simulink model "ElectricVehicleThermalManagementWithHeatPump"  (R2024b)
settings: Solver=VariableStepAuto  StartTime=0.0  StopTime=3600  RelTol=1e-3  AbsTol=1e-3
PreLoadFcn:
  | init_nmpc
InitFcn:
  | init_nmpc
model workspace: external: MATLAB File ElectricVehicleThermalManagementWithHeatPumpParameters.m (data not in the file)
values from neighbouring files (symbols this model uses):
  battery_C1_LUT = [1913.6 12447 30609 ... (first row only)    [ElectricVehicleThermalManagementWithHeatPumpParameters.m]
  battery_capacity_LUT = [280.081 276.25 276.392]    [ElectricVehicleThermalManagementWithHeatPumpParameters.m]
  battery_cell_cp = 795    [ElectricVehicleThermalManagementWithHeatPumpParameters.m]
  battery_cell_mass = 2.5    [ElectricVehicleThermalManagementWithHeatPumpParameters.m]
  battery_Em_LUT = [3.4966 3.5057 3.5148 ... (first row only)    [ElectricVehicleThermalManagementWithHeatPumpParameters.m]
  battery_N_cells = 20    [ElectricVehicleThermalManagementWithHeatPumpParameters.m]
  battery_Qe_init = 0    [ElectricVehicleThermalManagementWithHeatPumpParameters.m]
  battery_R0_LUT = [0.0117 0.0085 0.009 ... (first row only)    [ElectricVehicleThermalManagementWithHeatPumpParameters.m]
  battery_R1_LUT = [0.0109 0.0029 0.0013 ... (first row only)    [ElectricVehicleThermalManagementWithHeatPumpParameters.m]
  battery_SOC_LUT = [0; 0.1; 0.25; 0.5; 0.75; 0.9; 1]    [ElectricVehicleThermalManagementWithHeatPumpParameters.m]
  battery_T_init = -10    [ElectricVehicleThermalManagementWithHeatPumpParameters.m]
  battery_temperature_LUT = [5 20 40]    [ElectricVehicleThermalManagementWithHeatPumpParameters.m]
  cabin_duct_area = 0.04    [ElectricVehicleThermalManagementWithHeatPumpParameters.m]
  cabin_T_init = -10    [ElectricVehicleThermalManagementWithHeatPumpParameters.m]
  chiller_area_primary = 0.43982297150257105    (= 0.439822971503)    [ElectricVehicleThermalManagementWithHeatPumpParameters.m]
  chiller_N_baffles = 3    [ElectricVehicleThermalManagementWithHeatPumpParameters.m]
  chiller_N_tubes = 100    [ElectricVehicleThermalManagementWithHeatPumpParameters.m]
  chiller_tube_D = 0.0035    [ElectricVehicleThermalManagementWithHeatPumpParameters.m]
  chiller_tube_L = 0.4    [ElectricVehicleThermalManagementWithHeatPumpParameters.m]
  chiller_wall_conductivity = 240    [ElectricVehicleThermalManagementWithHeatPumpParameters.m]
  chiller_wall_thickness = 0.0001    [ElectricVehicleThermalManagementWithHeatPumpParameters.m]
  cond_evap_air_area_flow = 0.3906    [ElectricVehicleThermalManagementWithHeatPumpParameters.m]
  cond_evap_air_area_primary = 1.4834999999999998    (= 1.4835)    [ElectricVehicleThermalManagementWithHeatPumpParameters.m]
  cond_evap_W = 0.015    [ElectricVehicleThermalManagementWithHeatPumpParameters.m]
  cond_evap_wall_conductivity = 240    [ElectricVehicleThermalManagementWithHeatPumpParameters.m]
  cond_evap_wall_thickness = 0.0001    [ElectricVehicleThermalManagementWithHeatPumpParameters.m]
  coolant_channel_D = 0.0092    [ElectricVehicleThermalManagementWithHeatPumpParameters.m]
  coolant_pipe_D = 0.019    [ElectricVehicleThermalManagementWithHeatPumpParameters.m]
  coolant_T_init = -10    [ElectricVehicleThermalManagementWithHeatPumpParameters.m]
  coolant_tank_area = 0.0121    [ElectricVehicleThermalManagementWithHeatPumpParameters.m]
  coolant_tank_volume = 1.25    [ElectricVehicleThermalManagementWithHeatPumpParameters.m]
  coolant_valve_D_ratio_max = 0.95    [ElectricVehicleThermalManagementWithHeatPumpParameters.m]
  coolant_valve_D_ratio_min = 0.001    [ElectricVehicleThermalManagementWithHeatPumpParameters.m]
  coolant_valve_displacement = 0.0063    [ElectricVehicleThermalManagementWithHeatPumpParameters.m]
  coolant_valve_S_max = 0.0053    [ElectricVehicleThermalManagementWithHeatPumpParameters.m]
  evaporator_air_area_flow = 0.12    [ElectricVehicleThermalManagementWithHeatPumpParameters.m]
  evaporator_air_area_primary = 0.4323    [ElectricVehicleThermalManagementWithHeatPumpParameters.m]
  evaporator_W = 0.015    [ElectricVehicleThermalManagementWithHeatPumpParameters.m]
  evaporator_wall_conductivity = 240    [ElectricVehicleThermalManagementWithHeatPumpParameters.m]
  evaporator_wall_thickness = 0.0001    [ElectricVehicleThermalManagementWithHeatPumpParameters.m]
  expansion_valve_D_ratio_max = 0.9    [ElectricVehicleThermalManagementWithHeatPumpParameters.m]
  hex_area_primary = 0.070371675440411369    (= 0.0703716754404)    [ElectricVehicleThermalManagementWithHeatPumpParameters.m]
  hex_N_tubes = 64    [ElectricVehicleThermalManagementWithHeatPumpParameters.m]
  hex_tube_D = 0.0035    [ElectricVehicleThermalManagementWithHeatPumpParameters.m]
  hex_wall_conductivity = 240    [ElectricVehicleThermalManagementWithHeatPumpParameters.m]
  hex_wall_thickness = 0.0001    [ElectricVehicleThermalManagementWithHeatPumpParameters.m]
  inner_cond_air_area_flow = 0.1953    [ElectricVehicleThermalManagementWithHeatPumpParameters.m]
  inner_cond_air_area_primary = 0.99520000000000008    (= 0.9952)    [ElectricVehicleThermalManagementWithHeatPumpParameters.m]
  inner_cond_W = 0.02    [ElectricVehicleThermalManagementWithHeatPumpParameters.m]
  inner_cond_wall_conductivity = 240    [ElectricVehicleThermalManagementWithHeatPumpParameters.m]
  inner_cond_wall_thickness = 0.0001    [ElectricVehicleThermalManagementWithHeatPumpParameters.m]
  pump_speed_max = 1000    [ElectricVehicleThermalManagementWithHeatPumpParameters.m]
  radiator_air_area_flow = 0.097499999999999989    (= 0.0975)    [ElectricVehicleThermalManagementWithHeatPumpParameters.m]
  radiator_air_area_primary = 0.43687499999999996    (= 0.436875)    [ElectricVehicleThermalManagementWithHeatPumpParameters.m]
  radiator_W = 0.015    [ElectricVehicleThermalManagementWithHeatPumpParameters.m]
  radiator_wall_conductivity = 240    [ElectricVehicleThermalManagementWithHeatPumpParameters.m]
  radiator_wall_thickness = 0.0001    [ElectricVehicleThermalManagementWithHeatPumpParameters.m]
  refrigerant_p_init = 0.2    [ElectricVehicleThermalManagementWithHeatPumpParameters.m]
  refrigerant_pipe_D = 0.01    [ElectricVehicleThermalManagementWithHeatPumpParameters.m]
  refrigerant_valve_D_ratio_max = 0.95    [ElectricVehicleThermalManagementWithHeatPumpParameters.m]
  refrigerant_valve_displacement = 0.005    [ElectricVehicleThermalManagementWithHeatPumpParameters.m]
libraries: fl_lib x227, nesl_utility x162, SimscapeFluids_lib x30, LiBatteryElements_lib x16, slpidlib x3, SignalEditorBlockLib x1
(part 10 of 13)

== system ElectricVehicleThermalManagementWithHeatPump/Controls/Preview ==
  T_env : Inport
  Clock : Inport  Port=2
  Accleration : Constant  Value=|
      | [0
      | 0
      | 0
      | 0
      | 0
      | 0
      | 0
      | 0
      | 0
      | 0
      | 0
      | 0
      | 0
      | 0
      | 0
      | 4
      | 4
      | 1
      | 3
      | 2.50000000000000
      | 0.500000000000000
      | 0
      | 0
      | 0
      | 0
      | -0.500000000000000
      | -0.500000000000000
      | -1
      | -7
      | -6
      | 0
      | 0
      | 0
      | 0
      | 0
      | 0
      | 0
      | 0
      | 0
      | 0
      | 0
      | 0
      | 0
      | 0
      | 0
      | 0
      | 0
      | 0
      | 0
      | 0
      | 0
      | 0
      | 4
      | 4
      | 0
      | 1
      | 2.50000000000000
      | 2.50000000000000
      | 0.666666666666667
      | 1
      | 3.50000000000000
      | 4.50000000000000
      | 3
      | 2
      | 2
      | 0.500000000000000
      | 0
      | 0
      | 0
      | 0
      | 0
      | 0
      | 0
      | 0
      | 0
      | 0
      | 0
      | 0
      | 0
      | 0
      | 0
      | 0
      | -0.500000000000000
      | -0.500000000000000
      | 0
      | 0
      | 0
      | -0.500000000000000
      | -1.50000000000000
      | -2
      | -2.50000000000000
      | -2.50000000000000
      | -2.50000000000000
      | -2.50000000000000
      | -1.50000000000000
      | -8
      | -7.50000000000000
      | 0
      | 0
      | 0
      | 0
      | 0
      | 0
      | 0
      | 0
      | 0
      | 0
      | 0
      | 0
      | 0
      | 0
      | 0
      | 0
      | 0
      | 0
      | 0
      | 0
      | 0
      | 0
      | 3.50000000000000
      | 4
      | 0.500000000000000
      | 1
      | 3
      | 2.50000000000000
      | 0.333333333333333
      | 0.666666666666667
      | 2.50000000000000
      | 2.50000000000000
      | 2.50000000000000
      | 2.50000000000000
      | 2.50000000000000
      | 2
      | 1.50000000000000
      | 1.50000000000000
      | 1
      | 0.500000000000000
      | 1
      | 2.50000000000000
      | 2.50000000000000
      | 2
      | 1.50000000000000
      | 1.50000000000000
      | 1.50000000000000
      | 1
      | 1
      | 0.500000000000000
      | 0
      | 0
      | 0
      | 0
      | -0.500000000000000
      | -0.500000000000000
      | 0
      | 0
      | 0
      | -0.500000000000000
      | -1
      | -1.50000000000000
      | -2
      | -1.50000000000000
      | -1.50000000000000
      | -1.50000000000000
      | -1.50000000000000
      | -2
      | -0.500000000000000
      | 0
      | -0.500000000000000
      | 0
      | 0
      | 0
      | 0
      | 0
      | 0
      | 0
      | 0
      | 0
      | -0.666666666666667
      | -1
      | -2
      | -3
      | -3
      | -3
      | -3
      | -10
      | -8.50000000000000
      | 0
      | 0
      | 0
      | 0
      | 0
      | 0
      | 0
      | 0
      | 0
      | 0
      | 0
      | 0
      | 0
      | 0
      | 0
      | 0
      | 0
      | 0
      | 0
      | 0
      | 3
      | 4
      | 1
      | 1
      | 3
      | 2.50000000000000
      | 0.500000000000000
      | 0
      | 0
      | 0
      | 0
      | -0.500000000000000
      | -0.500000000000000
      | -1
      | -7
      | -6
      | 0
      | 0
      | 0
      | 0
      | 0
      | 0
      | 0
      | 0
      | 0
      | 0
      | 0
      | 0
      | 0
      | 0
      | 0
      | 0
      | 0
      | 0
      | 0
      | 0
      | 0
      | 0
      | 3
      | 4
      | 1
      | 1
      | 3
      | 2.50000000000000
      | 0.500000000000000
      | -0.500000000000000
      | 1.50000000000000
      | 4
      | 4
      | 3.50000000000000
      | 2.50000000000000
      | 1.50000000000000
      | 0.500000000000000
      | 0
      | 0
      | 0
      | 0
      | 0
      | 0
      | 0
      | 0
      | 0
      | 0
      | 0
      | 0
      | 0
      | 0
      | 0
      | 0
      | 0
      | -0.500000000000000
      | -0.500000000000000
      | 0
      | 0
      | -0.500000000000000
      | -1.50000000000000
      | -2
      | -2.50000000000000
      | -2.50000000000000
      | -2.50000000000000
      | -3
      | -9
      | -7.50000000000000
      | 0
      | 0
      | 0
      | 0
      | 0
      | 0
      | 0
      | 0
      | 0
      | 0
      | 0
      | 0
      | 0
      | 0
      | 0
      | 0
      | 0
      | 0
      | 0
      | 0
      | 0
      | 0
      | 0
      | 3
      | 3.50000000000000
      | 1
      | 1.50000000000000
      | 2.50000000000000
      | 2.50000000000000
      | 1.50000000000000
      | -0.500000000000000
      | 0.500000000000000
      | 3
      | 3
      | 2.50000000000000
      | 2
      | 2.50000000000000
      | 2.50000000000000
      | 2
      | 1
      | 0.333333333333333
      | 1
      | 2
      | 2
      | 2
      | 2
      | 1.50000000000000
      | 1.50000000000000
      | 1.50000000000000
      | 1
      | 0.500000000000000
      | 0
      | 0
      | 0
      | -0.500000000000000
      | 0
      | 0.500000000000000
      | -0.500000000000000
      | -0.500000000000000
      | 0
      | 0
      | -1
      | -2
      | -1.50000000000000
      | -1.50000000000000
      | -2
      | -2
      | -1.50000000000000
      | -1.50000000000000
      | -0.500000000000000
      | 0
      | -0.500000000000000
      | 0
      | 0
      | 0
      | 0
      | 0
      | 0
      | 0
      | 0
      | 0
      | -0.666666666666667
      | -1
      | -2
      | -3
      | -3
      | -3
      | -3
      | -10
      | -8.50000000000000
      | 0
      | 0
      | 0
      | 0
      | 0
      | 0
      | 0
      | 0
      | 0
      | 0
      | 0
      | 0
      | 0
      | 0
      | 0
      | 0
      | 0
      | 0
      | 0
      | 0
      | 3
      | 4
      | 1
      | 1
      | 3
      | 2.50000000000000
      | 0.500000000000000
      | 0
      | 0
      | 0
      | 0
      | -0.500000000000000
      | -0.500000000000000
      | -1
      | -7
      | -6
      | 0
      | 0
      | 0
      | 0
      | 0
      | 0
      | 0
      | 0
      | 0
      | 0
      | 0
      | 0
      | 0
      | 0
      | 0
      | 0
      | 0
      | 0
      | 0
      | 0
      | 0
      | 0
      | 3
      | 4
      | 1
      | 1
      | 2.50000000000000
      | 2.50000000000000
      | 1
      | -0.500000000000000
      | 1.50000000000000
      | 4.50000000000000
      | 4
      | 3
      | 2.50000000000000
      | 1.50000000000000
      | 0.500000000000000
      | 0
      | 0
      | 0
      | 0
      | 0
      | 0
      | 0
      | 0
      | 0
      | 0
      | 0
      | 0
      | 0
      | 0
      | 0
      | -0.500000000000000
      | 0
      | 0
      | -0.500000000000000
      | 0
      | 0
      | -0.500000000000000
      | -1.50000000000000
      | -2
      | -2.50000000000000
      | -2.50000000000000
      | -2.50000000000000
      | -3
      | -9
      | -7.50000000000000
      | 0
      | 0
      | 0
      | 0
      | 0
      | 0
      | 0
      | 0
      | 0
      | 0
      | 0
      | 0
      | 0
      | 0
      | 0
      | 0
      | 0
      | 0
      | 0
      | 0
      | 0
      | 0
      | 0
      | 3
      | 4
      | 1
      | 1
      | 2.50000000000000
      | 2.50000000000000
      | 1
      | 0
      | 1
      | 2
      | 3
      | 3
      | 2
      | 2
      | 2.50000000000000
      | 2.50000000000000
      | 1
      | 0.333333333333333
      | 1.33333333333333
      | 2.50000000000000
      | 2
      | 1.50000000000000
      | 1.50000000000000
      | 2
      | 1.50000000000000
      | 1
      | 1
      | 0.500000000000000
      | 0
      | 0
      | 0
      | 0
      | 0
      | -0.500000000000000
      | -0.500000000000000
      | 0
      | 0
      | 0
      | -1
      | -2
      | -1.50000000000000
      | -1.50000000000000
      | -2
      | -2
      | -1.50000000000000
      | -1.50000000000000
      | -1
      | 0
      | 0
      | 0
      | 0
      | 0
      | 0
      | 0
      | 0
      | 0
      | 0
      | 0
      | -0.666666666666667
      | -1
      | -2
      | -3
      | -3
      | -3
      | -3.50000000000000
      | -10
      | -8
      | 0
      | 0
      | 0
      | 0
      | 0
      | 0
      | 0
      | 0
      | 0
      | 0
      | 0
      | 0
      | 0
      | 0
      | 0
      | 0
      | 0
      | 0
      | 0
      | 0
      | 3
      | 4
      | 1
      | 1
      | 3
      | 2.50000000000000
      | 0.500000000000000
      | 0
      | 0
      | 0
      | 0
      | -0.500000000000000
      | -0.500000000000000
      | -1
      | -7
      | -6
      | 0
      | 0
      | 0
      | 0
      | 0
      | 0
      | 0
      | 0
      | 0
      | 0
      | 0
      | 0
      | 0
      | 0
      | 0
      | 0
      | 0
      | 0
      | 0
      | 0
      | 0
      | 0
      | 3
      | 4
      | 1
      | 1
      | 3
      | 2.50000000000000
      | 1
      | -0.500000000000000
      | 1
      | 4.50000000000000
      | 4
      | 3
      | 2.50000000000000
      | 1.50000000000000
      | 0.500000000000000
      | 0
      | 0
      | 0
      | 0
      | 0
      | 0
      | 0
      | 0
      | 0
      | 0
      | 0
      | 0
      | 0
      | 0
      | 0
      | 0
      | -0.500000000000000
      | -0.500000000000000
      | 0
      | 0
      | 0
      | -0.500000000000000
      | -1.50000000000000
      | -2.50000000000000
      | -2.50000000000000
      | -2
      | -2.50000000000000
      | -3
      | -9
      | -7.50000000000000
      | 0
      | 0
      | 0
      | 0
      | 0
      | 0
      | 0
      | 0
      | 0
      | 0
      | 0
      | 0
      | 0
      | 0
      | 0
      | 0
      | 0
      | 0
      | 0
      | 0
      | 0
      | 0
      | 0
      | 3
      | 3.50000000000000
      | 1
      | 1.50000000000000
      | 2.50000000000000
      | 2.50000000000000
      | 1
      | 0
      | 1
      | 2.50000000000000
      | 3
      | 2
      | 2.50000000000000
      | 3
      | 1.50000000000000
      | 2
      | 1.50000000000000
      | 0.333333333333333
      | 1
      | 2.50000000000000
      | 2
      | 2
      | 2
      | 1.50000000000000
      | 1.50000000000000
      | 1
      | 0.500000000000000
      | 0.500000000000000
      | 0.500000000000000
      | 0
      | 0
      | 0
      | 0
      | 0
      | 0
      | -0.500000000000000
      | -0.500000000000000
      | 0
      | -1
      | -2
      | -2
      | -1.50000000000000
      | -1
      | -1.50000000000000
      | -2
      | -2
      | -1
      | 0
      | 0
      | 0
      | 0
      | 0
      | 0
      | 0
      | 0
      | 0
      | 0
      | 0
      | -0.500000000000000
      | -1
      | -1
      | -2
      | -3
      | -3
      | -3
      | -3
      | -10
      | -8.50000000000000
      | 0
      | 0
      | 0
      | 0
      | 0
      | 0
      | 0
      | 0
      | 0
      | 0
      | 0
      | 0
      | 0
      | 0
      | 0
      | 0
      | 0
      | 0
      | 0
      | 0
      | 0
      | 0
      | 0
      | 0
      | 0
      | 0
      | 0
      | 0
      | 0
      | 3
      | 4
      | 1
      | 0.500000000000000
      | 1.50000000000000
      | 2.50000000000000
      | 2
      | 0.500000000000000
      | 1.50000000000000
      | 2
      | 2
      | 2
      | 2
      | 2.50000000000000
      | 2
      | 2
      | 2
      | 1
      | 1
      | 2
      | 2
      | 1.50000000000000
      | 1.50000000000000
      | 1.50000000000000
      | 1.50000000000000
      | 2
      | 1
      | 1
      | 2
      | 1
      | 1
      | 1.50000000000000
      | 1.50000000000000
      | 1.50000000000000
      | 1
      | 1.50000000000000
      | 2
      | 1.50000000000000
      | 1.50000000000000
      | 1
      | 0.333333333333333
      | 0.666666666666667
      | 0.500000000000000
      | -0.500000000000000
      | -0.500000000000000
      | 0
      | 0.500000000000000
      | 0
      | -0.500000000000000
      | 0
      | 0
      | 0
      | 0
      | 0
      | 0
      | 0
      | 0
      | 0.500000000000000
      | 0.500000000000000
      | -0.500000000000000
      | -0.500000000000000
      | 0.500000000000000
      | 0.500000000000000
      | -0.500000000000000
      | -0.500000000000000
      | 0
      | 0.500000000000000
      | 0.500000000000000
      | -0.500000000000000
      | 0
      | 0
      | -0.500000000000000
      | 0.500000000000000
      | 0
      | -0.500000000000000
      | 0.500000000000000
      | 0
      | -0.500000000000000
      | 0
      | 0
      | 0
      | 0.500000000000000
      | 0
      | -0.500000000000000
      | 0.500000000000000
      | 0.500000000000000
      | 0
      | -0.500000000000000
      | -1
      | -1.50000000000000
      | -2
      | -1.50000000000000
      | -2
      | -2.66666666666667
      | -2.50000000000000
      | -2.50000000000000
      | -1
      | 0
      | -0.500000000000000
      | 0
      | 0
      | 0
      | 0
      | 0
      | 0
      | 0
      | 0
      | 0
      | 0
      | 0
      | 0
      | 0
      | 0
      | 0
      | 0
      | 0
      | 0
      | 0
      | 0
      | 0
      | 0
      | 0
      | 0
      | 0
      | 0
      | 0
      | 0
      | 0
      | 0
      | 0
      | 0
      | 0
      | 0
      | 0
      | 0
      | 0
      | 0
      | 0
      | 0
      | 0
      | 0
      | 0
      | 0
      | 0
      | 0
      | 0
      | 0
      | 0
      | 0
      | 0
      | 0
      | 0
      | 0
      | 0
      | 0
      | 0
      | 0
      | 0
      | 0
      | 0
      | 0
      | 0
      | 0
      | 0
      | 0.500000000000000
      | 1
      | 1
      | 1.50000000000000
      | 1.50000000000000
      | 1.50000000000000
      | 2
      | 1
      | 1
      | 2
      | 1.50000000000000
      | 1
      | 1.50000000000000
      | 1
      | 0.333333333333333
      | 0.666666666666667
      | 0
      | -0.500000000000000
      | 0.500000000000000
      | 0.500000000000000
      | -0.500000000000000
      | -0.500000000000000
      | 0.500000000000000
      | 0.500000000000000
      | -0.500000000000000
      | 0
      | 0.500000000000000
      | 0
      | -0.500000000000000
      | -0.500000000000000
      | 0
      | 0
      | 0.500000000000000
      | 0
      | 0
      | 0.500000000000000
      | 0
      | 0
      | 0
      | 0
      | 0
      | -0.500000000000000
      | 0
      | 0.500000000000000
      | 0
      | 0
      | 0
      | -0.500000000000000
      | 0
      | 0.500000000000000
      | -0.500000000000000
      | 0
      | 0.500000000000000
      | 0
      | 0
      | 0
      | 0
      | 0
      | 0
      | 0
      | 0
      | 0
      | 0.500000000000000
      | 1
      | 1
      | 0.500000000000000
      | 1
      | 1
      | 0.500000000000000
      | 0.500000000000000
      | 0.500000000000000
      | 0.500000000000000
      | 0.500000000000000
      | 1
      | 1.50000000000000
      | 1.50000000000000
      | 0.500000000000000
      | 0.500000000000000
      | 1
      | 0.500000000000000
      | 0.500000000000000
      | 1.50000000000000
      | 1
      | 0
      | 0.500000000000000
      | 1.50000000000000
      | 1
      | 0.500000000000000
      | 1
      | 1
      | 1
      | 1
      | 1
      | 1
      | 0.500000000000000
      | 0.500000000000000
      | 0.500000000000000
      | 0.500000000000000
      | 0
      | 0
      | 1
      | 0.500000000000000
      | -0.500000000000000
      | 0
      | 0.500000000000000
      | 0
      | 0
      | 0
      | 0
      | -0.500000000000000
      | -0.500000000000000
      | 0.500000000000000
      | 0.500000000000000
      | 0
      | 0
      | -0.500000000000000
      | 0
      | 0.500000000000000
      | 0
      | 0
      | -0.500000000000000
      | 0
      | 0
      | 0
      | 0.500000000000000
      | 0.500000000000000
      | 0.500000000000000
      | -0.500000000000000
      | 1
      | 1.50000000000000
      | 1
      | 0.500000000000000
      | 0
      | 0.500000000000000
      | 1.50000000000000
      | 2
      | 0
      | 1
      | 1
      | 0
      | 1
      | 2
      | 2
      | 0.500000000000000
      | 0.500000000000000
      | 0.500000000000000
      | 0.500000000000000
      | 1.50000000000000
      | 0
      | -1
      | 0.500000000000000
      | 1
      | 0
      | -0.500000000000000
      | 0
      | 0
      | 0
      | -0.500000000000000
      | -2.50000000000000
      | -2.50000000000000
      | -1
      | -1.50000000000000
      | -2.50000000000000
      | -2.50000000000000
      | -2.50000000000000
      | -2.50000000000000
      | -2
      | -2
      | -2.50000000000000
      | -3
      | -3
      | -2.50000000000000
      | -2.50000000000000
      | -2.50000000000000
      | -3
      | -3.50000000000000
      | -3.50000000000000
      | -4
      | -3.50000000000000
      | -3.50000000000000
      | -4
      | -29
      | -27
      | 0
      | 0
      | 0
      | 0
      | 0
      | 0
      | 0
      | 0
      | 0
      | 0
      | 0
      | 0
      | 0
      | 0
      | 0
      | 0
      | 0
      | 0
      | 0
      | 0
      | 0
      | 0
      | 0
      | 0
      | 0
      | 0
      | 0
      | 0
      | 0
      | 0
      | 0
      | 0
      | 0
      | 0
      | 0
      | 0
      | 0
      | 0
      | 0
      | 0
      | 0
      | 0
      | 0
      | 0
      | 2.13114754098361
      | 0.0698924731182796
      | -0.0619047619047619
      | -0.240740740740741
      | 0]
  DCDC Heat vs Current : Lookup_n-D  NumberOfTableDimensions=1  BreakpointsForDimension1=[-100 0 25 50 300]  IndexSearchMethod=Linear search  BeginIndexSearchUsingPreviousIndexResult=on  Table=[250 0 40 70 400]  InternalRulePriority=Speed  RndMeth=Simplest
  Display : Display
  Inverter Current vs Acceleration : Lookup_n-D  NumberOfTableDimensions=1  BreakpointsForDimension1=[-10 -8 -5 0 5 8 10]  IndexSearchMethod=Linear search  BeginIndexSearchUsingPreviousIndexResult=on  Table=[200 150 100 0 100 150 200]*0.6  InternalRulePriority=Speed  RndMeth=Simplest
  Inverter Current vs Speed : Lookup_n-D  NumberOfTableDimensions=1  BreakpointsForDimension1=[0 60 80 100 120 140 160 180 200]  IndexSearchMethod=Linear search  BeginIndexSearchUsingPreviousIndexResult=on  Table=[0 10 18 27 45 65 100 120 160]  InternalRulePriority=Speed  RndMeth=Simplest
  Inverter Heat vs Current : Lookup_n-D  NumberOfTableDimensions=1  BreakpointsForDimension1=[-100 0 25 50 300]  IndexSearchMethod=Linear search  BeginIndexSearchUsingPreviousIndexResult=on  Table=[250 0 40 70 400]  InternalRulePriority=Speed  RndMeth=Simplest
  Motor Heat vs Current : Lookup_n-D  NumberOfTableDimensions=1  BreakpointsForDimension1=[-150 -70 -26 0 25 50 100 300 600]  IndexSearchMethod=Linear search  BeginIndexSearchUsingPreviousIndexResult=on  Table=[3500 2650 2100 0 400 550 4800 4800 4800]  InternalRulePriority=Speed  RndMeth=Simplest
  Saturation : Saturate  UpperLimit=200  LowerLimit=-inf  ZeroCross=off
  Speed : Constant  Value=|
      | [0
      | 0
      | 0
      | 0
      | 0
      | 0
      | 0
      | 0
      | 0
      | 0
      | 0
      | 0
      | 0
      | 0
      | 0
      | 0
      | 0
      | 8
      | 8
      | 10
      | 14
      | 15
      | 15
      | 15
      | 15
      | 15
      | 15
      | 14
      | 14
      | 12
      | 0
      | 0
      | 0
      | 0
      | 0
      | 0
      | 0
      | 0
      | 0
      | 0
      | 0
      | 0
      | 0
      | 0
      | 0
      | 0
      | 0
      | 0
      | 0
      | 0
      | 0
      | 0
      | 0
      | 0
      | 8
      | 8
      | 8
      | 10
      | 13
      | 15
      | 15
      | 18
      | 22
      | 27
      | 28
      | 31
      | 32
      | 32
      | 32
      | 32
      | 32
      | 32
      | 32
      | 32
      | 32
      | 32
      | 32
      | 32
      | 32
      | 32
      | 32
      | 32
      | 32
      | 32
      | 31
      | 31
      | 31
      | 31
      | 31
      | 30
      | 28
      | 26
      | 23
      | 21
      | 18
      | 16
      | 15
      | 0
      | 0
      | 0
      | 0
      | 0
      | 0
      | 0
      | 0
      | 0
      | 0
      | 0
      | 0
      | 0
      | 0
      | 0
      | 0
      | 0
      | 0
      | 0
      | 0
      | 0
      | 0
      | 0
      | 0
      | 7
      | 8
      | 8
      | 10
      | 14
      | 15
      | 15
      | 17
      | 20
      | 22
      | 25
      | 27
      | 30
      | 31
      | 33
      | 34
      | 35
      | 35
      | 37
      | 40
      | 42
      | 44
      | 45
      | 47
      | 48
      | 49
      | 50
      | 50
      | 50
      | 50
      | 50
      | 50
      | 49
      | 49
      | 49
      | 49
      | 49
      | 48
      | 47
      | 45
      | 43
      | 42
      | 40
      | 39
      | 37
      | 35
      | 36
      | 35
      | 35
      | 35
      | 35
      | 35
      | 35
      | 35
      | 35
      | 35
      | 35
      | 35
      | 33
      | 32
      | 29
      | 26
      | 23
      | 20
      | 17
      | 0
      | 0
      | 0
      | 0
      | 0
      | 0
      | 0
      | 0
      | 0
      | 0
      | 0
      | 0
      | 0
      | 0
      | 0
      | 0
      | 0
      | 0
      | 0
      | 0
      | 0
      | 0
      | 6
      | 8
      | 8
      | 10
      | 14
      | 15
      | 15
      | 15
      | 15
      | 15
      | 15
      | 14
      | 14
      | 12
      | 0
      | 0
      | 0
      | 0
      | 0
      | 0
      | 0
      | 0
      | 0
      | 0
      | 0
      | 0
      | 0
      | 0
      | 0
      | 0
      | 0
      | 0
      | 0
      | 0
      | 0
      | 0
      | 0
      | 0
      | 6
      | 8
      | 8
      | 10
      | 14
      | 15
      | 15
      | 14
      | 18
      | 22
      | 26
      | 29
      | 31
      | 32
      | 32
      | 32
      | 32
      | 32
      | 32
      | 32
      | 32
      | 32
      | 32
      | 32
      | 32
      | 32
      | 32
      | 32
      | 32
      | 32
      | 32
      | 32
      | 31
      | 31
      | 31
      | 31
      | 30
      | 28
      | 26
      | 23
      | 21
      | 18
      | 15
      | 0
      | 0
      | 0
      | 0
      | 0
      | 0
      | 0
      | 0
      | 0
      | 0
      | 0
      | 0
      | 0
      | 0
      | 0
      | 0
      | 0
      | 0
      | 0
      | 0
      | 0
      | 0
      | 0
      | 0
      | 0
      | 6
      | 7
      | 8
      | 10
      | 13
      | 15
      | 16
      | 14
      | 17
      | 20
      | 23
      | 25
      | 27
      | 30
      | 32
      | 34
      | 34
      | 35
      | 37
      | 39
      | 41
      | 43
      | 45
      | 46
      | 48
      | 49
      | 50
      | 50
      | 50
      | 50
      | 50
      | 49
      | 50
      | 50
      | 49
      | 49
      | 49
      | 49
      | 47
      | 45
      | 44
      | 42
      | 40
      | 38
      | 37
      | 35
      | 36
      | 35
      | 35
      | 35
      | 35
      | 35
      | 35
      | 35
      | 35
      | 35
      | 35
      | 35
      | 33
      | 32
      | 29
      | 26
      | 23
      | 20
      | 17
      | 0
      | 0
      | 0
      | 0
      | 0
      | 0
      | 0
      | 0
      | 0
      | 0
      | 0
      | 0
      | 0
      | 0
      | 0
      | 0
      | 0
      | 0
      | 0
      | 0
      | 0
      | 0
      | 6
      | 8
      | 8
      | 10
      | 14
      | 15
      | 15
      | 15
      | 15
      | 15
      | 15
      | 14
      | 14
      | 12
      | 0
      | 0
      | 0
      | 0
      | 0
      | 0
      | 0
      | 0
      | 0
      | 0
      | 0
      | 0
      | 0
      | 0
      | 0
      | 0
      | 0
      | 0
      | 0
      | 0
      | 0
      | 0
      | 0
      | 0
      | 6
      | 8
      | 8
      | 10
      | 13
      | 15
      | 15
      | 14
      | 18
      | 23
      | 26
      | 29
      | 31
      | 32
      | 32
      | 32
      | 32
      | 32
      | 32
      | 32
      | 32
      | 32
      | 32
      | 32
      | 32
      | 32
      | 32
      | 32
      | 32
      | 32
      | 31
      | 32
      | 31
      | 31
      | 31
      | 31
      | 30
      | 28
      | 26
      | 23
      | 21
      | 18
      | 15
      | 0
      | 0
      | 0
      | 0
      | 0
      | 0
      | 0
      | 0
      | 0
      | 0
      | 0
      | 0
      | 0
      | 0
      | 0
      | 0
      | 0
      | 0
      | 0
      | 0
      | 0
      | 0
      | 0
      | 0
      | 0
      | 6
      | 8
      | 8
      | 10
      | 13
      | 15
      | 15
      | 15
      | 17
      | 19
      | 23
      | 25
      | 27
      | 29
      | 32
      | 34
      | 34
      | 35
      | 38
      | 40
      | 42
      | 43
      | 45
      | 47
      | 48
      | 49
      | 50
      | 50
      | 50
      | 50
      | 50
      | 50
      | 50
      | 49
      | 49
      | 49
      | 49
      | 49
      | 47
      | 45
      | 44
      | 42
      | 40
      | 38
      | 37
      | 35
      | 35
      | 35
      | 35
      | 35
      | 35
      | 35
      | 35
      | 35
      | 35
      | 35
      | 35
      | 35
      | 33
      | 32
      | 29
      | 26
      | 23
      | 20
      | 16
      | 0
      | 0
      | 0
      | 0
      | 0
      | 0
      | 0
      | 0
      | 0
      | 0
      | 0
      | 0
      | 0
      | 0
      | 0
      | 0
      | 0
      | 0
      | 0
      | 0
      | 0
      | 0
      | 6
      | 8
      | 8
      | 10
      | 14
      | 15
      | 15
      | 15
      | 15
      | 15
      | 15
      | 14
      | 14
      | 12
      | 0
      | 0
      | 0
      | 0
      | 0
      | 0
      | 0
      | 0
      | 0
      | 0
      | 0
      | 0
      | 0
      | 0
      | 0
      | 0
      | 0
      | 0
      | 0
      | 0
      | 0
      | 0
      | 0
      | 0
      | 6
      | 8
      | 8
      | 10
      | 14
      | 15
      | 16
      | 14
      | 18
      | 23
      | 26
      | 29
      | 31
      | 32
      | 32
      | 32
      | 32
      | 32
      | 32
      | 32
      | 32
      | 32
      | 32
      | 32
      | 32
      | 32
      | 32
      | 32
      | 32
      | 32
      | 32
      | 31
      | 31
      | 31
      | 31
      | 31
      | 30
      | 28
      | 25
      | 23
      | 21
      | 18
      | 15
      | 0
      | 0
      | 0
      | 0
      | 0
      | 0
      | 0
      | 0
      | 0
      | 0
      | 0
      | 0
      | 0
      | 0
      | 0
      | 0
      | 0
      | 0
      | 0
      | 0
      | 0
      | 0
      | 0
      | 0
      | 0
      | 6
      | 7
      | 8
      | 10
      | 13
      | 15
      | 15
      | 15
      | 17
      | 20
      | 23
      | 24
      | 28
      | 30
      | 31
      | 34
      | 34
      | 35
      | 37
      | 40
      | 41
      | 44
      | 45
      | 47
      | 48
      | 49
      | 49
      | 50
      | 50
      | 50
      | 50
      | 50
      | 50
      | 50
      | 50
      | 49
      | 49
      | 49
      | 47
      | 45
      | 43
      | 42
      | 41
      | 39
      | 37
      | 35
      | 35
      | 35
      | 35
      | 35
      | 35
      | 35
      | 35
      | 35
      | 35
      | 35
      | 35
      | 35
      | 34
      | 33
      | 32
      | 29
      | 26
      | 23
      | 20
      | 17
      | 0
      | 0
      | 0
      | 0
      | 0
      | 0
      | 0
      | 0
      | 0
      | 0
      | 0
      | 0
      | 0
      | 0
      | 0
      | 0
      | 0
      | 0
      | 0
      | 0
      | 0
      | 0
      | 0
      | 0
      | 0
      | 0
      | 0
      | 0
      | 0
      | 0
      | 0
      | 6
      | 8
      | 8
      | 9
      | 11
      | 14
      | 15
      | 15
      | 18
      | 19
      | 22
      | 23
      | 26
      | 28
      | 30
      | 32
      | 34
      | 35
      | 37
      | 39
      | 41
      | 42
      | 44
      | 45
      | 47
      | 49
      | 50
      | 52
      | 54
      | 54
      | 56
      | 57
      | 59
      | 60
      | 61
      | 63
      | 65
      | 66
      | 68
      | 68
      | 69
      | 70
      | 70
      | 69
      | 69
      | 69
      | 70
      | 69
      | 69
      | 69
      | 69
      | 69
      | 69
      | 69
      | 69
      | 69
      | 69
      | 70
      | 70
      | 69
      | 69
      | 70
      | 70
      | 69
      | 69
      | 69
      | 70
      | 70
      | 69
      | 70
      | 69
      | 69
      | 70
      | 69
      | 69
      | 70
      | 69
      | 69
      | 69
      | 69
      | 69
      | 70
      | 69
      | 69
      | 70
      | 70
      | 70
      | 69
      | 68
      | 66
      | 64
      | 63
      | 58
      | 55
      | 53
      | 50
      | 51
      | 50
      | 50
      | 50
      | 50
      | 50
      | 50
      | 50
      | 50
      | 50
      | 50
      | 50
      | 50
      | 50
      | 50
      | 50
      | 50
      | 50
      | 50
      | 50
      | 50
      | 50
      | 50
      | 50
      | 50
      | 50
      | 50
      | 50
      | 50
      | 50
      | 50
      | 50
      | 50
      | 50
      | 50
      | 50
      | 50
      | 50
      | 50
      | 50
      | 50
      | 50
      | 50
      | 50
      | 50
      | 50
      | 50
      | 50
      | 50
      | 50
      | 50
      | 50
      | 50
      | 50
      | 50
      | 50
      | 50
      | 50
      | 50
      | 50
      | 50
      | 50
      | 50
      | 50
      | 50
      | 50
      | 50
      | 50
      | 51
      | 52
      | 53
      | 55
      | 56
      | 58
      | 60
      | 60
      | 62
      | 64
      | 65
      | 66
      | 68
      | 68
      | 69
      | 70
      | 69
      | 69
      | 70
      | 70
      | 69
      | 69
      | 70
      | 70
      | 69
      | 70
      | 70
      | 70
      | 69
      | 69
      | 69
      | 69
      | 70
      | 69
      | 70
      | 70
      | 70
      | 70
      | 70
      | 70
      | 70
      | 69
      | 70
      | 70
      | 70
      | 70
      | 70
      | 69
      | 70
      | 70
      | 69
      | 70
      | 70
      | 70
      | 70
      | 70
      | 70
      | 70
      | 70
      | 70
      | 70
      | 70
      | 71
      | 72
      | 73
      | 73
      | 75
      | 75
      | 76
      | 76
      | 77
      | 77
      | 78
      | 79
      | 81
      | 82
      | 82
      | 83
      | 84
      | 84
      | 85
      | 87
      | 87
      | 87
      | 88
      | 90
      | 90
      | 91
      | 92
      | 93
      | 94
      | 95
      | 96
      | 97
      | 97
      | 98
      | 98
      | 99
      | 98
      | 99
      | 100
      | 100
      | 99
      | 100
      | 100
      | 100
      | 100
      | 100
      | 100
      | 99
      | 99
      | 100
      | 100
      | 100
      | 100
      | 99
      | 100
      | 100
      | 100
      | 100
      | 99
      | 100
      | 99
      | 100
      | 100
      | 101
      | 101
      | 100
      | 103
      | 103
      | 105
      | 104
      | 105
      | 105
      | 108
      | 109
      | 108
      | 111
      | 110
      | 111
      | 112
      | 115
      | 116
      | 116
      | 117
      | 117
      | 118
      | 120
      | 118
      | 118
      | 119
      | 120
      | 119
      | 119
      | 119
      | 119
      | 119
      | 118
      | 114
      | 113
      | 112
      | 110
      | 107
      | 105
      | 102
      | 100
      | 98
      | 96
      | 93
      | 90
      | 87
      | 85
      | 82
      | 80
      | 76
      | 73
      | 69
      | 65
      | 62
      | 58
      | 54
      | 0
      | 0
      | 0
      | 0
      | 0
      | 0
      | 0
      | 0
      | 0
      | 0
      | 0
      | 0
      | 0
      | 0
      | 0
      | 0
      | 0
      | 0
      | 0
      | 0
      | 0
      | 0
      | 0
      | 0
      | 0
      | 0
      | 0
      | 0
      | 0
      | 0
      | 0
      | 0
      | 0
      | 0
      | 0
      | 0
      | 0
      | 0
      | 0
      | 0
      | 0
      | 0
      | 0
      | 0
      | 0
      | 0
      | 130
      | 130
      | 0]
  SpeedPreview : MATLAB Function  TreatAsAtomicUnit=on
  Sum : Sum  Inputs=|++
  condEvapAirFlow2 : MATLAB Function  TreatAsAtomicUnit=on
  time : Constant  Value=|
      | [1
      | 2
      | 3
      | 4
      | 5
      | 6
      | 7
      | 8
      | 9
      | 10
      | 11
      | 12
      | 13
      | 14
      | 15
      | 16
      | 17
      | 18
      | 19
      | 20
      | 21
      | 22
      | 23
      | 24
      | 25
      | 26
      | 27
      | 28
      | 29
      | 30
      | 31
      | 32
      | 33
      | 34
      | 35
      | 36
      | 37
      | 38
      | 39
      | 40
      | 41
      | 42
      | 43
      | 44
      | 45
      | 46
      | 47
      | 48
      | 49
      | 50
      | 51
      | 52
      | 53
      | 54
      | 55
      | 56
      | 57
      | 58
      | 59
      | 61
      | 62
      | 63
      | 64
      | 65
      | 66
      | 67
      | 68
      | 69
      | 70
      | 71
      | 72
      | 73
      | 74
      | 75
      | 76
      | 77
      | 78
      | 79
      | 80
      | 81
      | 82
      | 83
      | 84
      | 85
      | 86
      | 87
      | 88
      | 89
      | 90
      | 91
      | 92
      | 93
      | 94
      | 95
      | 96
      | 97
      | 98
      | 99
      | 100
      | 101
      | 102
      | 103
      | 104
      | 105
      | 106
      | 107
      | 108
      | 109
      | 110
      | 111
      | 112
      | 113
      | 114
      | 115
      | 116
      | 117
      | 118
      | 119
      | 120
      | 121
      | 122
      | 123
      | 124
      | 125
      | 126
      | 127
      | 129
      | 130
      | 131
      | 132
      | 133
      | 134
      | 135
      | 136
      | 137
      | 138
      | 139
      | 140
      | 141
      | 142
      | 143
      | 144
      | 145
      | 146
      | 147
      | 148
      | 149
      | 150
      | 151
      | 152
      | 153
      | 154
      | 155
      | 156
      | 157
      | 158
      | 159
      | 160
      | 161
      | 162
      | 163
      | 164
      | 165
      | 166
      | 167
      | 168
      | 169
      | 170
      | 171
      | 172
      | 173
      | 174
      | 175
      | 176
      | 177
      | 178
      | 179
      | 180
      | 182
      | 183
      | 184
      | 185
      | 186
      | 187
      | 188
      | 189
      | 190
      | 191
      | 192
      | 193
      | 194
      | 195
      | 196
      | 197
      | 198
      | 199
      | 200
      | 201
      | 202
      | 203
      | 204
      | 205
      | 206
      | 207
      | 208
      | 209
      | 210
      | 211
      | 212
      | 213
      | 214
      | 215
      | 216
      | 217
      | 218
      | 219
      | 220
      | 221
      | 222
      | 223
      | 224
      | 225
      | 226
      | 227
      | 228
      | 229
      | 230
      | 231
      | 232
      | 233
      | 234
      | 235
      | 236
      | 237
      | 238
      | 239
      | 240
      | 241
      | 242
      | 243
      | 244
      | 245
      | 246
      | 247
      | 248
      | 249
      | 250
      | 251
      | 252
      | 253
      | 254
      | 255
      | 256
      | 257
      | 258
      | 259
      | 260
      | 261
      | 262
      | 263
      | 264
      | 265
      | 266
      | 267
      | 268
      | 269
      | 270
      | 271
      | 272
      | 273
      | 274
      | 275
      | 276
      | 277
      | 278
      | 279
      | 280
      | 281
      | 282
      | 283
      | 284
      | 285
      | 286
      | 287
      | 288
      | 289
      | 290
      | 291
      | 292
      | 293
      | 294
      | 295
      | 296
      | 297
      | 298
      | 299
      | 300
      | 301
      | 302
      | 303
      | 304
      | 305
      | 306
      | 307
      | 308
      | 309
      | 310
      | 311
      | 312
      | 313
      | 314
      | 315
      | 316
      | 317
      | 318
      | 319
      | 320
      | 321
      | 322
      | 323
      | 324
      | 325
      | 326
      | 327
      | 328
      | 329
      | 330
      | 331
      | 332
      | 333
      | 335
      | 336
      | 337
      | 338
      | 339
      | 340
      | 341
      | 342
      | 343
      | 344
      | 345
      | 346
      | 347
      | 348
      | 349
      | 350
      | 351
      | 352
      | 353
      | 354
      | 355
      | 356
      | 357
      | 358
      | 359
      | 360
      | 361
      | 362
      | 363
      | 364
      | 365
      | 366
      | 367
      | 368
      | 369
      | 370
      | 371
      | 372
      | 373
      | 374
      | 375
      | 377
      | 378
      | 379
      | 380
      | 381
      | 382
      | 383
      | 384
      | 385
      | 386
      | 387
      | 388
      | 389
      | 390
      | 391
      | 392
      | 393
      | 394
      | 395
      | 396
      | 397
      | 398
      | 399
      | 400
      | 401
      | 402
      | 403
      | 404
      | 405
      | 406
      | 407
      | 408
      | 409
      | 410
      | 411
      | 412
      | 413
      | 414
      | 415
      | 416
      | 417
      | 418
      | 419
      | 420
      | 421
      | 422
      | 423
      | 424
      | 425
      | 426
      | 427
      | 428
      | 429
      | 430
      | 431
      | 432
      | 433
      | 434
      | 435
      | 436
      | 437
      | 438
      | 439
      | 440
      | 441
      | 442
      | 443
      | 444
      | 445
      | 446
      | 447
      | 448
      | 449
      | 450
      | 451
      | 452
      | 453
      | 454
      | 455
      | 456
      | 457
      | 458
      | 459
      | 460
      | 461
      | 462
      | 463
      | 464
      | 465
      | 466
      | 467
      | 468
      | 469
      | 470
      | 471
      | 472
      | 473
      | 474
      | 475
      | 476
      | 477
      | 478
      | 479
      | 480
      | 481
      | 482
      | 483
      | 484
      | 485
      | 486
      | 487
      | 488
      | 489
      | 490
      | 491
      | 492
      | 493
      | 494
      | 495
      | 496
      | 497
      | 498
      | 499
      | 500
      | 501
      | 502
      | 503
      | 504
      | 505
      | 506
      | 507
      | 508
      | 509
      | 510
      | 511
      | 512
      | 513
      | 514
      | 515
      | 516
      | 517
      | 518
      | 519
      | 520
      | 521
      | 522
      | 523
      | 524
      | 525
      | 526
      | 527
      | 528
      | 530
      | 531
      | 532
      | 533
      | 534
      | 535
      | 536
      | 537
      | 538
      | 539
      | 540
      | 541
      | 542
      | 543
      | 544
      | 545
      | 546
      | 547
      | 548
      | 549
      | 550
      | 551
      | 552
      | 553
      | 554
      | 555
      | 556
      | 557
      | 558
      | 559
      | 560
      | 561
      | 562
      | 563
      | 564
      | 565
      | 566
      | 567
      | 568
      | 569
      | 570
      | 572
      | 573
      | 574
      | 575
      | 576
      | 577
      | 578
      | 579
      | 580
      | 581
      | 582
      | 583
      | 584
      | 585
      | 586
      | 587
      | 588
      | 589
      | 590
      | 591
      | 592
      | 593
      | 594
      | 595
      | 596
      | 597
      | 598
      | 599
      | 600
      | 601
      | 602
      | 603
      | 604
      | 605
      | 606
      | 607
      | 608
      | 609
      | 610
      | 611
      | 612
      | 613
      | 614
      | 615
      | 616
      | 617
      | 618
      | 619
      | 620
      | 621
      | 622
      | 623
      | 624
      | 625
      | 626
      | 627
      | 628
      | 629
      | 630
      | 631
      | 632
      | 633
      | 634
      | 635
      | 636
      | 637
      | 638
      | 639
      | 640
      | 641
      | 642
      | 643
      | 644
      | 645
      | 646
      | 647
      | 648
      | 649
      | 650
      | 651
      | 652
      | 653
      | 654
      | 655
      | 656
      | 657
      | 658
      | 659
      | 660
      | 661
      | 662
      | 663
      | 664
      | 665
      | 666
      | 667
      | 668
      | 669
      | 670
      | 671
      | 672
      | 673
      | 674
      | 675
      | 676
      | 677
      | 678
      | 679
      | 680
      | 681
      | 682
      | 683
      | 684
      | 685
      | 686
      | 687
      | 688
      | 689
      | 690
      | 691
      | 692
      | 693
      | 694
      | 695
      | 696
      | 697
      | 698
      | 699
      | 700
      | 701
      | 702
      | 703
      | 704
      | 705
      | 706
      | 707
      | 708
      | 709
      | 710
      | 711
      | 712
      | 713
      | 714
      | 715
      | 716
      | 717
      | 718
      | 719
      | 720
      | 721
      | 722
      | 723
      | 725
      | 726
      | 727
      | 728
      | 729
      | 730
      | 731
      | 732
      | 733
      | 734
      | 735
      | 736
      | 737
      | 738
      | 739
      | 740
      | 741
      | 742
      | 743
      | 744
      | 745
      | 746
      | 747
      | 748
      | 749
      | 750
      | 751
      | 752
      | 753
      | 754
      | 755
      | 756
      | 757
      | 758
      | 759
      | 760
      | 761
      | 762
      | 763
      | 764
      | 765
      | 766
      | 767
      | 768
      | 769
      | 770
      | 771
      | 772
      | 773
      | 774
      | 775
      | 776
      | 777
      | 778
      | 779
      | 780
      | 781
      | 782
      | 783
      | 784
      | 785
      | 786
      | 787
      | 788
      | 789
      | 790
      | 791
      | 792
      | 793
      | 794
      | 795
      | 796
      | 797
      | 798
      | 799
      | 800
      | 801
      | 802
      | 803
      | 804
      | 805
      | 806
      | 807
      | 808
      | 809
      | 810
      | 811
      | 812
      | 813
      | 814
      | 815
      | 816
      | 817
      | 818
      | 819
      | 820
      | 821
      | 823
      | 824
      | 825
      | 826
      | 827
      | 828
      | 829
      | 830
      | 831
      | 833
      | 834
      | 835
      | 836
      | 837
      | 838
      | 839
      | 840
      | 841
      | 842
      | 843
      | 844
      | 845
      | 846
      | 848
      | 849
      | 850
      | 851
      | 852
      | 853
      | 854
      | 855
      | 856
      | 857
      | 858
      | 859
      | 860
      | 861
      | 862
      | 863
      | 864
      | 865
      | 866
      | 867
      | 868
      | 869
      | 870
      | 871
      | 872
      | 873
      | 874
      | 875
      | 876
      | 877
      | 878
      | 879
      | 880
      | 881
      | 882
      | 883
      | 884
      | 885
      | 886
      | 887
      | 888
      | 889
      | 890
      | 891
      | 892
      | 893
      | 894
      | 895
      | 896
      | 897
      | 898
      | 899
      | 901
      | 902
      | 903
      | 904
      | 905
      | 906
      | 907
      | 908
      | 909
      | 910
      | 911
      | 912
      | 913
      | 914
      | 915
      | 916
      | 917
      | 918
      | 919
      | 920
      | 921
      | 922
      | 923
      | 924
      | 925
      | 926
      | 927
      | 928
      | 929
      | 930
      | 931
      | 932
      | 933
      | 934
      | 935
      | 936
      | 937
      | 938
      | 939
      | 940
      | 941
      | 942
      | 943
      | 944
      | 945
      | 946
      | 947
      | 948
      | 949
      | 950
      | 951
      | 952
      | 953
      | 954
      | 955
      | 956
      | 957
      | 958
      | 959
      | 960
      | 961
      | 962
      | 963
      | 964
      | 965
      | 966
      | 967
      | 968
      | 969
      | 970
      | 971
      | 972
      | 973
      | 974
      | 975
      | 976
      | 977
      | 978
      | 979
      | 980
      | 981
      | 982
      | 983
      | 984
      | 985
      | 986
      | 988
      | 989
      | 990
      | 991
      | 992
      | 993
      | 994
      | 995
      | 996
      | 997
      | 998
      | 999
      | 1000
      | 1001
      | 1002
      | 1003
      | 1004
      | 1005
      | 1006
      | 1007
      | 1008
      | 1009
      | 1010
      | 1011
      | 1012
      | 1013
      | 1014
      | 1015
      | 1016
      | 1017
      | 1018
      | 1019
      | 1020
      | 1021
      | 1022
      | 1023
      | 1024
      | 1025
      | 1026
      | 1027
      | 1028
      | 1029
      | 1030
      | 1031
      | 1032
      | 1033
      | 1034
      | 1035
      | 1036
      | 1037
      | 1038
      | 1039
      | 1040
      | 1041
      | 1042
      | 1043
      | 1044
      | 1045
      | 1046
      | 1047
      | 1048
      | 1049
      | 1050
      | 1051
      | 1052
      | 1053
      | 1054
      | 1055
      | 1056
      | 1057
      | 1058
      | 1059
      | 1060
      | 1061
      | 1062
      | 1063
      | 1064
      | 1065
      | 1066
      | 1067
      | 1068
      | 1069
      | 1070
      | 1071
      | 1072
      | 1073
      | 1074
      | 1075
      | 1076
      | 1077
      | 1078
      | 1079
      | 1080
      | 1081
      | 1082
      | 1083
      | 1084
      | 1085
      | 1086
      | 1087
      | 1088
      | 1089
      | 1090
      | 1091
      | 1092
      | 1093
      | 1094
      | 1095
      | 1096
      | 1097
      | 1098
      | 1099
      | 1100
      | 1101
      | 1102
      | 1103
      | 1104
      | 1105
      | 1106
      | 1107
      | 1108
      | 1109
      | 1110
      | 1111
      | 1112
      | 1113
      | 1114
      | 1115
      | 1116
      | 1117
      | 1118
      | 1119
      | 1120
      | 1121
      | 1122
      | 1123
      | 1124
      | 1125
      | 1126
      | 1127
      | 1128
      | 1129
      | 1130
      | 1131
      | 1132
      | 1133
      | 1134
      | 1135
      | 1136
      | 1137
      | 1138
      | 1139
      | 1140
      | 1141
      | 1142
      | 1143
      | 1144
      | 1145
      | 1146
      | 1147
      | 1148
      | 1149
      | 1150
      | 1151
      | 1152
      | 1153
      | 1154
      | 1155
      | 1156
      | 1157
      | 1158
      | 1159
      | 1160
      | 1161
      | 1162
      | 1163
      | 1164
      | 1165
      | 1166
      | 1167
      | 1168
      | 1169
      | 1170
      | 1171
      | 1172
      | 1173
      | 1174
      | 1175
      | 1176
      | 1177
      | 1178
      | 1179
      | 1180
      | 1181
      | 1182
      | 1183
      | 1184
      | 1185
      | 1186
      | 1187
      | 1188
      | 1189
      | 1190
      | 1191
      | 1192
      | 1193
      | 1194
      | 1195
      | 1196
      | 1197
      | 1198
      | 1199
      | 1200
      | 1260
      | 3060
      | 3360
      | 3600]
  Tenv : Outport
  MotHeat : Outport  Port=2
  InvHeat : Outport  Port=3
  DCDCHeat : Outport  Port=4
  BatteryCurrent : Outport  Port=5
  speed : Outport  Port=6
  mfCondEvap : Outport  Port=7
  wires:
  Inverter Current vs Acceleration/1 -> Sum/2
  Inverter Current vs Speed/1 -> Sum/1
  Accleration/1 -> SpeedPreview/4(a_grid)
  Saturation/1 -> Motor Heat vs Current/1, DCDC Heat vs Current/1, Inverter Heat vs Current/1, BatteryCurrent/1  "BatteryCurrent"
  time/1 -> SpeedPreview/2(t_grid)
  Sum/1 -> Saturation/1
  SpeedPreview/2(a_vec) -> Inverter Current vs Acceleration/1
  Clock/1 -> SpeedPreview/1(t)
  Speed/1 -> SpeedPreview/3(v_grid)
  Inverter Heat vs Current/1 -> InvHeat/1  "InvHeat"
  Motor Heat vs Current/1 -> MotHeat/1  "MotHeat"
  DCDC Heat vs Current/1 -> DCDCHeat/1  "DCDCHeat"
  T_env/1 -> SpeedPreview/5(tenv)
  SpeedPreview/3(Tenv_vec) -> Tenv/1
  SpeedPreview/1(v_vec) -> condEvapAirFlow2/1(speed), speed/1, Inverter Current vs Speed/1, Display/1
  condEvapAirFlow2/1(mfCondEvap) -> mfCondEvap/1
